simulink model "motor_movement"  (R2025b)
settings: Solver=FixedStepAuto  StartTime=0.0  StopTime=inf  RelTol=1e-3  EnableMultiTasking=on
libraries: raspberrypiBasiclib x5, raspberrypiNetworklib x1
settings Model: ExtModeTrigDuration=2  Creator=sport  LastModifiedBy=sport
settings SolverCC: PositivePriorityOrder=on
settings OptimizationCC: EnhancedBackFolding=on  PassReuseOutputArgsAs=Individual arguments  ZeroExternalMemoryAtStartup=off  ZeroInternalMemoryAtStartup=off  MaxStackSize=200000  OptimizeBlockOrder=speed  DifferentSizesBufferReuse=on  OptimizationCustomize=off  EfficientTunableParamExpr=on
settings DebuggingCC: ParameterTunabilityLossMsg=error
settings HardwareCC: ProdBitPerPointer=32.0  ProdBitPerSizeT=32.0  ProdBitPerPtrDiffT=32.0  ProdLargestAtomicInteger=Long  ProdLargestAtomicFloat=Double  ProdWordSize=32.0  ProdLongLongMode=on  ProdHWDeviceType=ARM Compatible->ARM Cortex-A (32-bit)
settings RTWCC: SystemTargetFile=ert.tlc  HardwareBoard=Raspberry Pi  TLCOptions="-aInlineSetEventsForThisBaseRateFcn=TLC_FALSE -aSuppressMultiTaskScheduler=TLC_FALSE  -aRateBasedStepFcn=0"  TemplateMakefile=ert_default_tmf  Toolchain=GNU GCC Embedded Linux  BuildConfiguration=Faster Runs  Description=Embedded Coder
settings CodeAppCC: ForceParamTrailComments=on  IgnoreCustomStorageClasses=off  OperatorAnnotations=on  SimulinkDataObjDesc=on  SFDataObjDesc=on  InsertBlockDesc=on
settings ERTTargetCC: ExtModeTransport=2.0  ExtModeStaticAlloc=on  ExtModeMexFile=ext_xcp  ExtModeIntrfLevel=Level2 - Open  InlinedParameterPlacement=Hierarchical  CodeReplacementLibrary=ARM Cortex-A CMSIS  SupportVariableSizeSignals=on

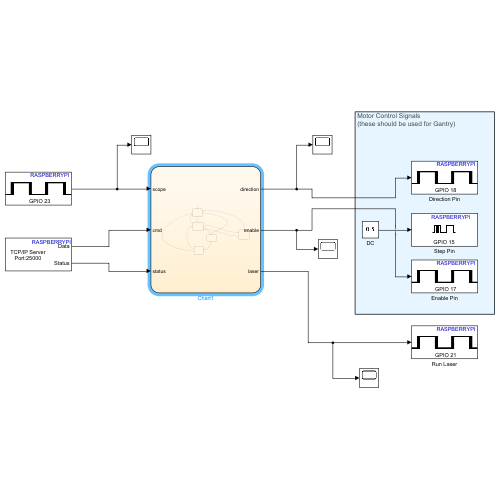
[thumbnail: Simulink's stored preview of the top-level diagram]
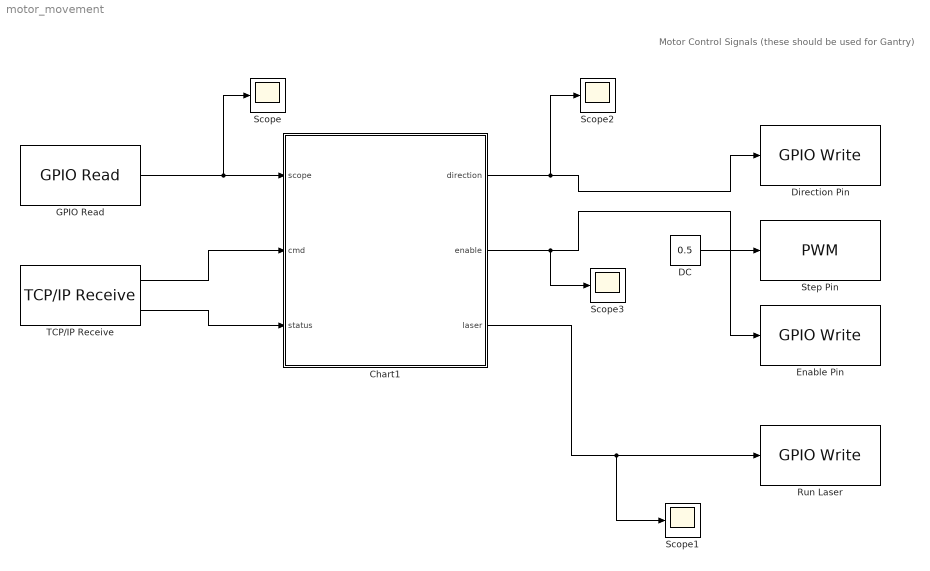
== system motor_movement ==
  note: Motor Control Signals
      | (these should be used for Gantry)
  Chart1 : Stateflow chart  TreatAsAtomicUnit=on
  DC : Constant  Value=0.5  VectorParams1D=off  SampleTime=-1
  Direction Pin : raspberrypiBasiclib/GPIO Write  BoardProperty=Pi 3 Model B+  gpio=18  blockPlatform=Raspberry Pi  PinNumber=17  board=[]  direction=[]
  Enable Pin : raspberrypiBasiclib/GPIO Write  BoardProperty=Pi 3 Model B+  gpio=17  blockPlatform=Raspberry Pi  PinNumber=17  board=[]  direction=[]
  GPIO Read : raspberrypiBasiclib/GPIO Read  BoardProperty=Pi 3 Model B+  gpio=23  SampleTime=-1  blockPlatform=Raspberry Pi  PinNumber=4  board=[]  direction=[]  internalResistor=[]
  Run Laser : raspberrypiBasiclib/GPIO Write  BoardProperty=Pi 3 Model B+  gpio=21  blockPlatform=Raspberry Pi  PinNumber=17  board=[]  direction=[]
  Scope{,1..3} (4 alike) : Scope
      Scope settings: ActiveDisplayYMinimum=-31.209230355781681  ActiveDisplayYMaximum=27.412853381835138
      Scope1 settings: ActiveDisplayYMinimum=-2.7680411559203213  ActiveDisplayYMaximum=2.76410690507973
      Scope2 settings: ActiveDisplayYMinimum=-112.80842815268726  ActiveDisplayYMaximum=89.7594706605618  DataLoggingVariableName=ScopeData2
      Scope3 settings: ActiveDisplayYMinimum=-641.555542250552  ActiveDisplayYMaximum=526.55309017332115  DataLoggingVariableName=ScopeData3
  Step Pin : raspberrypiBasiclib/PWM  board=Pi 3 Model B+  Pin_=15  Frequency=1000  blockPlatform=Raspberry Pi
  TCP/IP Receive : raspberrypiNetworklib/TCP//IP Receive  Mode_=Server  LocalServerPort_=25000  RemoteAddr_=127.0.0.1  RemoteServerPort_=25000  DataType_=uint8  DataSize_=1  SampleTime_=0.01  SimulateUsing=Code generation  ClientPortBindingSelection_=off  ClientPortToBind_=35000  BlockingMode_=off  BlockTimeout_=0.1  BlockPlatform=RASPBERRYPI
  wires:
  TCP/IP Receive/1 -> Chart1/2(cmd)
  DC/1 -> Step Pin/1
  GPIO Read/1 -> Chart1/1(scope), Scope/1
  Chart1/1(direction) -> Scope2/1, Direction Pin/1
  Chart1/2(enable) -> Scope3/1, Enable Pin/1
  TCP/IP Receive/2 -> Chart1/3(status)
  Chart1/3(laser) -> Scope1/1, Run Laser/1

== stateflow chart motor_movement/Chart1 ==
  state Start
    en:
    n=0;
    enable = 1;
    direction = 1;
    laser = 0;
  state Forward
    en:
    enable=0;
    direction=1;
    laser = 0;
    du:
    n = n + 1;
  state Home
    en:
    enable = 0;
    direction = 0;
    laser = 0;
    du:
    n = n - 1;
  state Shoot
    en:
    enable=1;
    laser = 1;
    ex:
    laser = 0;
  state Off
    en:
    enable=1;
    direction=0,
  state Backward
    en:
    enable = 0;
    direction = 0;
    laser = 0;
    du:
    n = n - 1
  (default) -> Start
  Home -> Start [order 1] : [status == 1 && cmd == 0]
  Shoot -> Start [order 2] : [status == 1 && cmd == 0]
  Home -> Start [order 2] : [n <=0]
  Backward -> Start [order 2] : [status == 1 && cmd == 0]
  Off -> Start [order 2] : [status == 1 && cmd == 0]
  Forward -> Start [order 2] : [status == 1 && cmd == 0]
  Start -> Forward : [scope == 1 && cmd == 1 && status == 1]
  Forward -> Home [order 4] : [status == 1 && cmd == 3]
  Backward -> Forward [order 1] : [after(8, sec)]
  Forward -> Shoot [order 3] : [status == 1 && cmd == 2]
  Shoot -> Forward [order 1] : [after(2, sec)]
  Forward -> Off [order 1] : [scope==0]
  Off -> Backward [order 1] : [after(2, sec)]
  data: direction output; enable output; scope input; cmd input; status input; laser output; n local =0
